simulink model "Acrobot_SingleAnglePD"  (R2025b)
settings: Solver=ode45  StartTime=0.0  StopTime=Tstop  MaxStep=1e-3  RelTol=1e-7  AbsTol=1e-9
values from neighbouring files (symbols this model uses):
  j_meas = g(1)    [run_simulink_models.m]
  Kd = g(3)    [run_simulink_models.m]
  Kp = g(2)    [run_simulink_models.m]
  qs = [pi; 0]    [make_simulink_figures.m]    (also in run_simulink_models.m = cases{r, 2})
  x0 = [deg2rad(3); 0; 0; 0]    [make_simulink_figures.m]    (also in run_simulink_models.m = [deg2rad(d0); 0; 0])
settings Model: Creator=bhargav_vemparala  LastModifiedBy=bhargav_vemparala

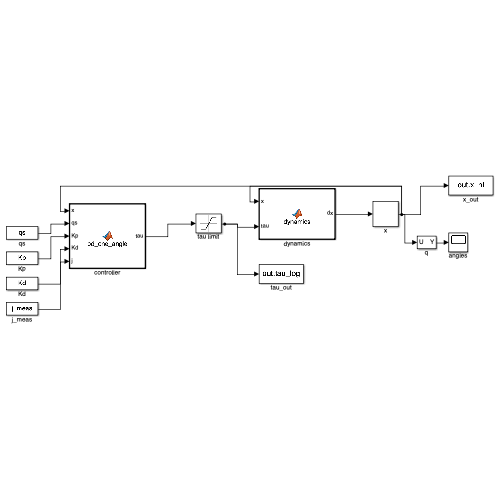
[thumbnail: Simulink's stored preview of the top-level diagram]
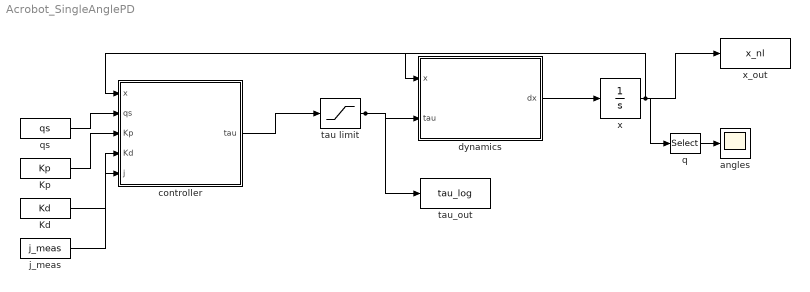
== system Acrobot_SingleAnglePD ==
  Kd : Constant  Value=Kd
  Kp : Constant  Value=Kp
  angles : Scope
  controller : MATLAB Function  TreatAsAtomicUnit=on
  dynamics : MATLAB Function  TreatAsAtomicUnit=on
  j_meas : Constant  Value=j_meas
  q : Selector  InputPortWidth=4  IndexOptions=Index vector (dialog)  Indices=[1 2]  OutputSizes=1
  qs : Constant  Value=qs
  tau limit : Saturate  UpperLimit=20  LowerLimit=-20
  tau_out : ToWorkspace  VariableName=tau_log  SaveFormat=Timeseries  SampleTime=-1
  x : Integrator  InitialCondition=x0
  x_out : ToWorkspace  VariableName=x_nl  SaveFormat=Timeseries  SampleTime=-1
  wires:
  dynamics/1(dx) -> x/1
  x/1 -> dynamics/1(x), x_out/1, q/1, controller/1(x)
  tau limit/1 -> dynamics/2(tau), tau_out/1
  q/1 -> angles/1
  qs/1 -> controller/2(qs)
  Kp/1 -> controller/3(Kp)
  Kd/1 -> controller/4(Kd)
  j_meas/1 -> controller/5(j)
  controller/1(tau) -> tau limit/1

== matlab function Acrobot_SingleAnglePD/controller ==
  data: x input; tau output; qs input; Kp input; Kd input; j input
function tau = pd_one_angle(x, qs, Kp, Kd, j)
%#codegen
% PD on ONE measured joint angle: tau = -(Kp e + Kd e_dot)
e = mod(x(j) - qs(j) + pi, 2*pi) - pi;
tau = -(Kp*e + Kd*x(j + 2));

== matlab function Acrobot_SingleAnglePD/dynamics ==
  data: x input; dx output; tau input
function dx = dynamics(x, tau)
%#codegen
% Given acrobot model: M(q) qdd + C(q,qd) qd = tau_g(q) + B tau
q1 = x(1); q2 = x(2); d1 = x(3); d2 = x(4);
c2 = cos(q2); s2 = sin(q2);
M = [2.663 + 2*c2, 1.33 + c2; 1.33 + c2, 1.33];
Cqd = [-s2*(2*d1*d2 + d2^2); s2*d1^2];
tg = -9.81*[1.5*sin(q1) + sin(q1 + q2); sin(q1 + q2)];
qdd = M \ (tg + [0; tau] - Cqd);
dx = [d1; d2; qdd(1); qdd(2)];
